simulink model "v5_2025_11_26_D2_rate_adaptive_revised"  (R2025a)
settings: Solver=FixedStepAuto  StartTime=0.0  StopTime=inf  FixedStep=1e-3  RelTol=1e-3  EnableMultiTasking=on
undefined symbols (not defined in the file): A0, A1, D0, D1, D10, D11, D12, D13, D2, D3, D4, D5, D6, D7, D8, D9, PTA0, PTA1, PTA2, PTB2, PTB23, PTB3, PTB9, PTC16, PTC17, PTC2, PTC3, PTC4, PTD0, PTD1, PTD2, PTD3
libraries: frdmk64flib x18, etargetslib x2, dspstat3 x1
settings Model: ExtModeTrigDuration=5  Creator=School Account  LastModifiedBy=zhang
settings SolverCC: AlgebraicLoopSolver=TrustRegion
settings OptimizationCC: DefaultParameterBehavior=Inlined  EnhancedBackFolding=on  PassReuseOutputArgsAs=Individual arguments  ZeroExternalMemoryAtStartup=off  ZeroInternalMemoryAtStartup=off  MaxStackSize=64  OptimizeBlockOrder=speed  DifferentSizesBufferReuse=on  OptimizationCustomize=off  EfficientTunableParamExpr=on
settings DebuggingCC: ParameterTunabilityLossMsg=error
settings HardwareCC: ProdBitPerPointer=32.0  ProdBitPerSizeT=32.0  ProdBitPerPtrDiffT=32.0  ProdLargestAtomicInteger=Long  ProdLargestAtomicFloat=Double  ProdWordSize=32.0  ProdHWDeviceType=ARM Compatible->ARM Cortex
settings SFSimCC: MATLABDynamicMemAlloc=off
settings RTWCC: SystemTargetFile=ert.tlc  HardwareBoard=NXP FRDM-K64F  TLCOptions="-aInlineSetEventsForThisBaseRateFcn=TLC_FALSE -aSuppressMultiTaskScheduler=TLC_FALSE  -aRateBasedStepFcn=0"  TemplateMakefile=ert_default_tmf  Toolchain=GNU Tools for ARM Embedded Processors  GPUComputeCapability=3.5  Description=Embedded Coder
settings CodeAppCC: ForceParamTrailComments=on  IgnoreCustomStorageClasses=off  OperatorAnnotations=on  SimulinkDataObjDesc=on  SFDataObjDesc=on  InsertBlockDesc=on
settings ERTTargetCC: ExtModeTransport=4.0  ExtModeStaticAlloc=off  ExtModeMexFile=sendToCommService  ExtModeIntrfLevel=Level1  DynamicArrayContainerType=coder::array

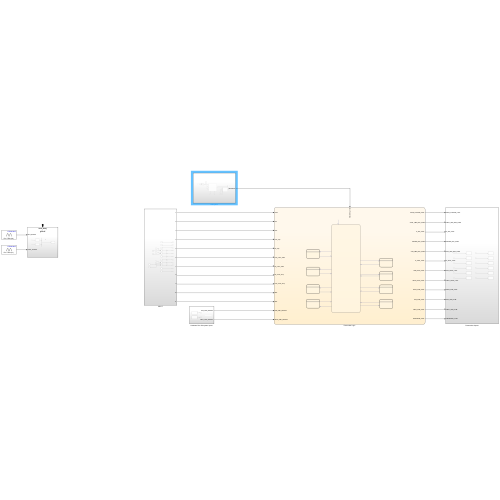
[thumbnail: Simulink's stored preview of the top-level diagram]
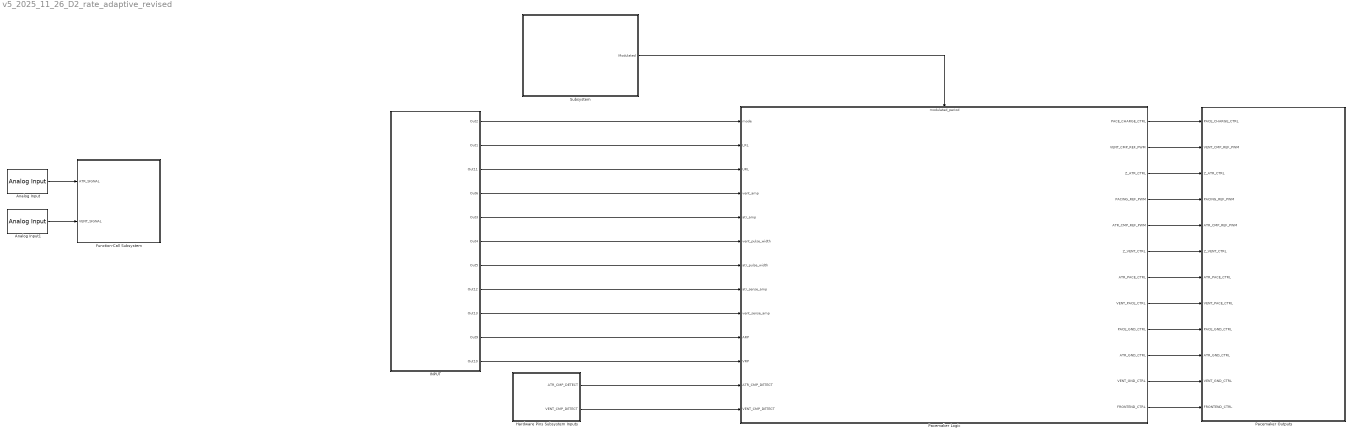
== system v5_2025_11_26_D2_rate_adaptive_revised ==
  Analog Input : frdmk64flib/Analog Input  Whichpin=PTB2 (A0)  SampleTime=-1
  Analog Input1 : frdmk64flib/Analog Input  Whichpin=PTB3 (A1)  SampleTime=-1
  Function-Call Subsystem : Subsystem  TreatAsAtomicUnit=on
  Hardware Pins Subsystem Inputs : Subsystem
  "INPUT " : Subsystem
  Pacemaker Logic : Stateflow chart  TreatAsAtomicUnit=on
      settings: PortSchema="{\"entries\":[{\"content\":{\"sides\":[{\"content\":{\"connectorIds\":[\"In1\",\"In4\",\"In13\",\"In5\",\"In2\",\"In6\",\"In3\",\"In7\",\"In10\",\"In8\",\"In11\",\"In9\",\"In12\"]},\"type\":\"ConnectorPlacement.EquallySpacedRectSide\",\"uuid\":\"2821f65a-9b3e-4ca7-babd-b0602bfdca31\"},{\"content\":{\"connectorIds\":[\"Out1\",\"Out2\",\"Out3\",\"Out4\",\"Out5\",\"Out6\",\"Out7\",\"Out8\",\"Out9\",\"Out10\",\"Out11\",\"Out12\"],\"side\":\"RIGHT\"},\"type\":\"ConnectorPlacement.EquallySpacedRectSide\",\"uuid\":\"3302ad84-7e85-4bae-9388-240b69681e7f\"},{\"content\":{\"connectorIds\":[\"In14\"],\"side\":\"TOP\"},\"type\":\"ConnectorPlacement.EquallySpacedRectSide\",\"uuid\":\"cc666da6-1c79-42dc-9f95-9791247ae8bf\"},{\"content\":{\"side\":\"BOTTOM\"},\"type\":\"ConnectorPlacement.EquallySpacedRectSide\",\"uuid\":\"6c7eefe5-bab4-42c2-8766-4f3cee9532f0\"}]},\"type\":\"ConnectorPlacement.EquallySpacedConnector\",\"uuid\":\"e2a43bfa-d126-4f35-adbf-2cf33da0501f\"}],\"packageUris\":[\"http://schema.mathworks.com/mf0/Connector/R2020b\"],\"version\":\"1.0\"}"
  Pacemaker Outputs : Subsystem
  Subsystem : Subsystem
  wires:
  Pacemaker Logic/1(PACE_CHARGE_CTRL) -> Pacemaker Outputs/1(PACE_CHARGE_CTRL)
  Pacemaker Logic/3(Z_ATR_CTRL) -> Pacemaker Outputs/3(Z_ATR_CTRL)
  Pacemaker Logic/4(PACING_REF_PWM) -> Pacemaker Outputs/4(PACING_REF_PWM)
  Pacemaker Logic/7(ATR_PACE_CTRL) -> Pacemaker Outputs/7(ATR_PACE_CTRL)
  Pacemaker Logic/9(PACE_GND_CTRL) -> Pacemaker Outputs/9(PACE_GND_CTRL)
  Pacemaker Logic/10(ATR_GND_CTRL) -> Pacemaker Outputs/10(ATR_GND_CTRL)
  Pacemaker Logic/11(VENT_GND_CTRL) -> Pacemaker Outputs/11(VENT_GND_CTRL)
  Pacemaker Logic/8(VENT_PACE_CTRL) -> Pacemaker Outputs/8(VENT_PACE_CTRL)
  Pacemaker Logic/6(Z_VENT_CTRL) -> Pacemaker Outputs/6(Z_VENT_CTRL)
  Pacemaker Logic/12(FRONTEND_CTRL) -> Pacemaker Outputs/12(FRONTEND_CTRL)
  Pacemaker Logic/5(ATR_CMP_REF_PWM) -> Pacemaker Outputs/5(ATR_CMP_REF_PWM)
  Pacemaker Logic/2(VENT_CMP_REF_PWM) -> Pacemaker Outputs/2(VENT_CMP_REF_PWM)
  Hardware Pins Subsystem Inputs/2(VENT_CMP_DETECT) -> Pacemaker Logic/12(VENT_CMP_DETECT)
  Hardware Pins Subsystem Inputs/1(ATR_CMP_DETECT) -> Pacemaker Logic/9(ATR_CMP_DETECT)
  "INPUT "/10(Out9) -> Pacemaker Logic/8(ARP)
  "INPUT "/11(Out10) -> Pacemaker Logic/11(VRP)
  "INPUT "/9(Out13) -> Pacemaker Logic/10(vent_sense_amp)
  "INPUT "/8(Out12) -> Pacemaker Logic/7(atr_sense_amp)
  "INPUT "/7(Out5) -> Pacemaker Logic/3(atr_pulse_width)
  "INPUT "/6(Out4) -> Pacemaker Logic/6(vent_pulse_width)
  "INPUT "/5(Out3) -> Pacemaker Logic/2(atr_amp)
  "INPUT "/4(Out6) -> Pacemaker Logic/5(vent_amp)
  "INPUT "/1(Out2) -> Pacemaker Logic/1(mode)
  "INPUT "/2(Out1) -> Pacemaker Logic/4(LRL)
  "INPUT "/3(Out11) -> Pacemaker Logic/13(URL)
  Analog Input/1 -> Function-Call Subsystem/1(ATR_SIGNAL)
  Analog Input1/1 -> Function-Call Subsystem/2(VENT_SIGNAL)
  Subsystem/1(Modulated) -> Pacemaker Logic/14(modulated_period)

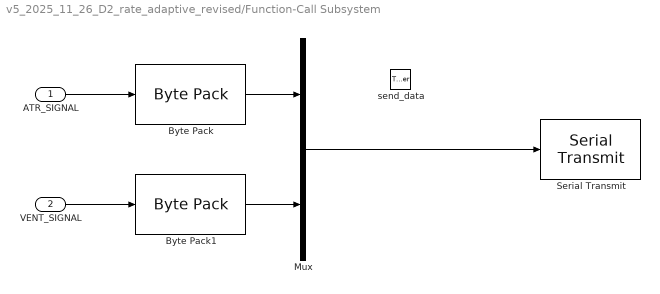
== system v5_2025_11_26_D2_rate_adaptive_revised/Function-Call Subsystem ==
  ATR_SIGNAL : Inport
  VENT_SIGNAL : Inport  Port=2
  send_data : TriggerPort  TriggerType=function-call  IsSimulinkFunction=on  FunctionName=send_data  VariantControl=(inherit)
  Byte Pack : etargetslib/Byte Pack  datatypes={'double'}  byteAlign=1
  Byte Pack1 : etargetslib/Byte Pack  datatypes={'double'}  byteAlign=1
  Mux : Mux  Inputs=2
  Serial Transmit : frdmk64flib/Serial Transmit  SCIModule=0  Baudrate=uint32(9600)  Parity=None  StopBits=1  HardwareFlowControl=None  ByteOrder=LittleEndian  BlockingMode=on  OutputStatus=off
  wires:
  ATR_SIGNAL/1 -> Byte Pack/1
  VENT_SIGNAL/1 -> Byte Pack1/1
  Byte Pack/1 -> Mux/1
  Mux/1 -> Serial Transmit/1
  Byte Pack1/1 -> Mux/2

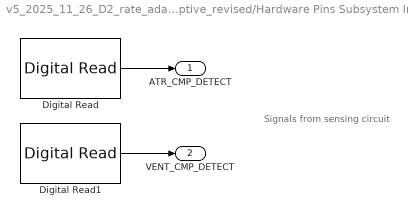
== system v5_2025_11_26_D2_rate_adaptive_revised/Hardware Pins Subsystem Inputs ==
  note: Signals from sensing circuit
  Digital Read : frdmk64flib/Digital Read  Whichpin=PTC16 (D0)  SampleTime=-1
  Digital Read1 : frdmk64flib/Digital Read  Whichpin=PTC17 (D1)  SampleTime=-1
  ATR_CMP_DETECT : Outport
  VENT_CMP_DETECT : Outport  Port=2
  wires:
  Digital Read1/1 -> VENT_CMP_DETECT/1
  Digital Read/1 -> ATR_CMP_DETECT/1

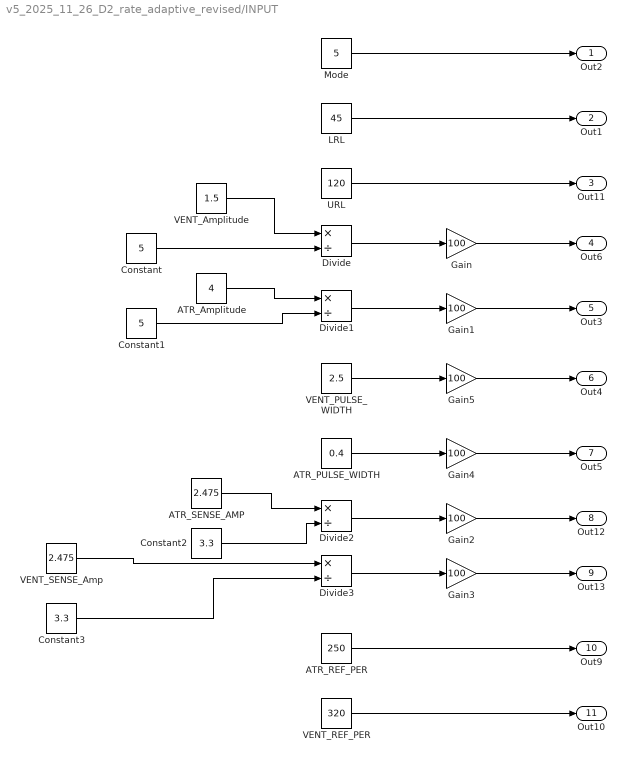
== system v5_2025_11_26_D2_rate_adaptive_revised/INPUT  ==
  ATR_Amplitude : Constant  Value=4
  ATR_PULSE_WIDTH : Constant  Value=0.4
  ATR_REF_PER : Constant  Value=250
  ATR_SENSE_AMP : Constant  Value=2.475
  Constant : Constant  Value=5
  Constant1 : Constant  Value=5
  Constant2 : Constant  Value=3.3
  Constant3 : Constant  Value=3.3
  Divide{,1..3} (4 alike) : Product  Inputs=*/
  Gain{,1..5} (6 alike) : Gain  Gain=100
  LRL : Constant  Value=45
  Mode : Constant  Value=5
  URL : Constant  Value=120
  VENT_Amplitude : Constant  Value=1.5
  VENT_PULSE_WIDTH : Constant  Value=2.5
  VENT_REF_PER : Constant  Value=320
  VENT_SENSE_Amp : Constant  Value=2.475
  Out2 : Outport
  Out1 : Outport  Port=2
  Out11 : Outport  Port=3
  Out6 : Outport  Port=4
  Out3 : Outport  Port=5
  Out4 : Outport  Port=6
  Out5 : Outport  Port=7
  Out12 : Outport  Port=8
  Out13 : Outport  Port=9
  Out9 : Outport  Port=10
  Out10 : Outport  Port=11
  wires:
  LRL/1 -> Out1/1
  URL/1 -> Out11/1
  Mode/1 -> Out2/1
  ATR_REF_PER/1 -> Out9/1
  VENT_REF_PER/1 -> Out10/1
  VENT_Amplitude/1 -> Divide/1
  Gain/1 -> Out6/1
  ATR_Amplitude/1 -> Divide1/1
  Gain1/1 -> Out3/1
  ATR_SENSE_AMP/1 -> Divide2/1
  Gain2/1 -> Out12/1
  VENT_SENSE_Amp/1 -> Divide3/1
  Gain3/1 -> Out13/1
  VENT_PULSE_WIDTH/1 -> Gain5/1
  Gain5/1 -> Out4/1
  ATR_PULSE_WIDTH/1 -> Gain4/1
  Gain4/1 -> Out5/1
  Divide/1 -> Gain/1
  Constant/1 -> Divide/2
  Divide1/1 -> Gain1/1
  Constant1/1 -> Divide1/2
  Divide2/1 -> Gain2/1
  Constant2/1 -> Divide2/2
  Divide3/1 -> Gain3/1
  Constant3/1 -> Divide3/2

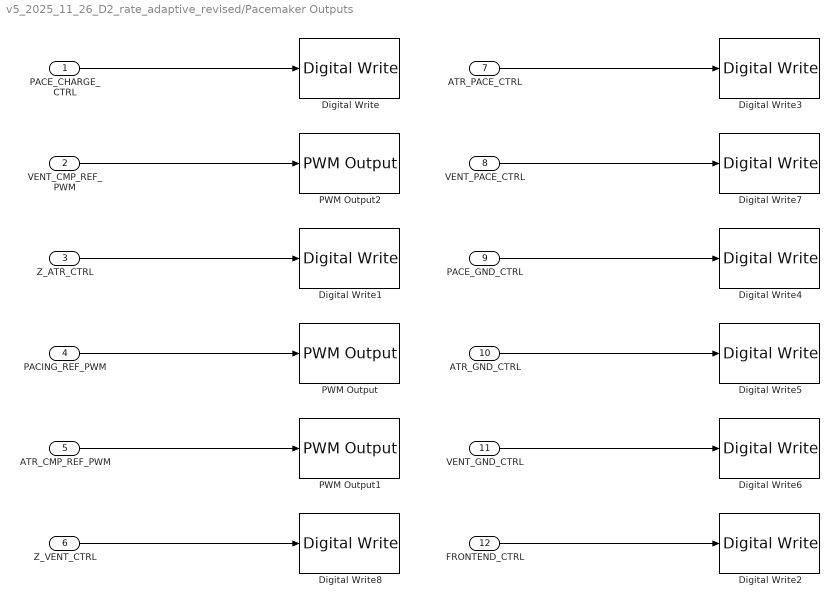
== system v5_2025_11_26_D2_rate_adaptive_revised/Pacemaker Outputs ==
  PACE_CHARGE_CTRL : Inport
  VENT_CMP_REF_PWM : Inport  Port=2
  Z_ATR_CTRL : Inport  Port=3
  PACING_REF_PWM : Inport  Port=4
  ATR_CMP_REF_PWM : Inport  Port=5
  Z_VENT_CTRL : Inport  Port=6
  ATR_PACE_CTRL : Inport  Port=7
  VENT_PACE_CTRL : Inport  Port=8
  PACE_GND_CTRL : Inport  Port=9
  ATR_GND_CTRL : Inport  Port=10
  VENT_GND_CTRL : Inport  Port=11
  FRONTEND_CTRL : Inport  Port=12
  Digital Write : frdmk64flib/Digital Write  Whichpin=PTB9 (D2)
  Digital Write1 : frdmk64flib/Digital Write  Whichpin=PTB23 (D4)
  Digital Write2 : frdmk64flib/Digital Write  Whichpin=PTD1 (D13)
  Digital Write3 : frdmk64flib/Digital Write  Whichpin=PTA0 (D8)
  Digital Write4 : frdmk64flib/Digital Write  Whichpin=PTD0 (D10)
  Digital Write5 : frdmk64flib/Digital Write  Whichpin=PTD2 (D11)
  Digital Write6 : frdmk64flib/Digital Write  Whichpin=PTD3 (D12)
  Digital Write7 : frdmk64flib/Digital Write  Whichpin=PTC4 (D9)
  Digital Write8 : frdmk64flib/Digital Write  Whichpin=PTC3 (D7)
  PWM Output : frdmk64flib/PWM Output  Whichpin=PTA2 (D5)  InitialFrequency=2000  InitialDutyCycle=0
  PWM Output1 : frdmk64flib/PWM Output  Whichpin=PTC2 (D6)  InitialFrequency=2000  InitialDutyCycle=0
  PWM Output2 : frdmk64flib/PWM Output  Whichpin=PTA1 (D3)  InitialFrequency=2000  InitialDutyCycle=0
  wires:
  PACE_CHARGE_CTRL/1 -> Digital Write/1
  Z_ATR_CTRL/1 -> Digital Write1/1
  PACING_REF_PWM/1 -> PWM Output/1
  ATR_PACE_CTRL/1 -> Digital Write3/1
  PACE_GND_CTRL/1 -> Digital Write4/1
  ATR_GND_CTRL/1 -> Digital Write5/1
  VENT_GND_CTRL/1 -> Digital Write6/1
  VENT_PACE_CTRL/1 -> Digital Write7/1
  Z_VENT_CTRL/1 -> Digital Write8/1
  FRONTEND_CTRL/1 -> Digital Write2/1
  ATR_CMP_REF_PWM/1 -> PWM Output1/1
  VENT_CMP_REF_PWM/1 -> PWM Output2/1

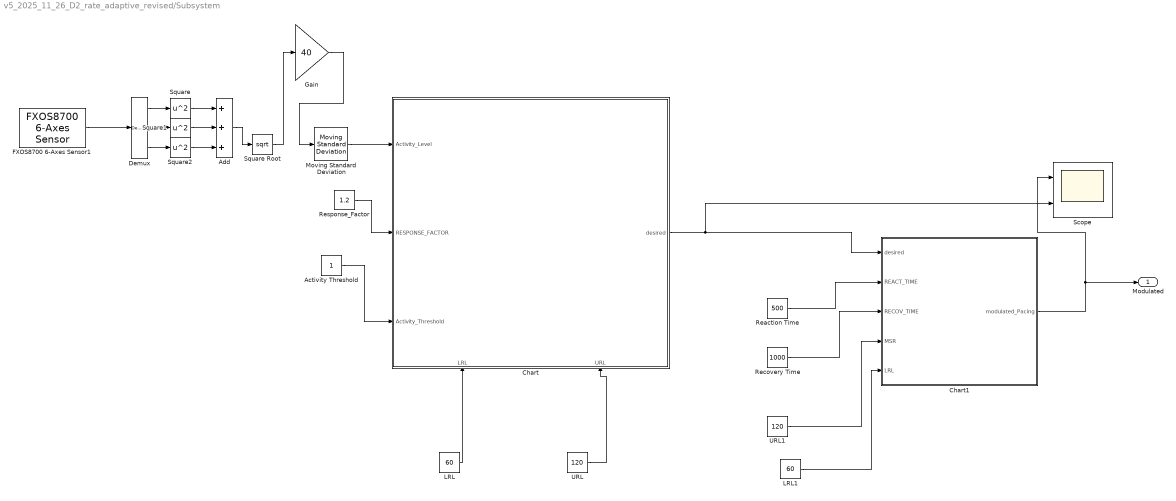
== system v5_2025_11_26_D2_rate_adaptive_revised/Subsystem ==
  Activity Threshold : Constant
  Add : Sum  Inputs=+++
  Chart : Stateflow chart  TreatAsAtomicUnit=on
      settings: PortSchema="{\"entries\":[{\"content\":{\"sides\":[{\"content\":{\"connectorIds\":[\"In3\",\"In4\",\"In5\"]},\"type\":\"ConnectorPlacement.EquallySpacedRectSide\",\"uuid\":\"74c786d3-d2a6-437e-8bb7-c9d9b4a74617\"},{\"content\":{\"connectorIds\":[\"Out1\"],\"side\":\"RIGHT\"},\"type\":\"ConnectorPlacement.EquallySpacedRectSide\",\"uuid\":\"2c46704d-1ce5-4a26-9635-57e0f6503ead\"},{\"content\":{\"side\":\"TOP\"},\"type\":\"ConnectorPlacement.EquallySpacedRectSide\",\"uuid\":\"1e7c0bb1-a8b6-49e0-9e63-e8e48adc5546\"},{\"content\":{\"connectorIds\":[\"In1\",\"In2\"],\"side\":\"BOTTOM\"},\"type\":\"ConnectorPlacement.EquallySpacedRectSide\",\"uuid\":\"98fe2a4d-8dd5-42bc-97d4-b5234350e537\"}]},\"type\":\"ConnectorPlacement.EquallySpacedConnector\",\"uuid\":\"114a6ead-843c-4291-bcbc-4dc58f15d580\"}],\"packageUris\":[\"http://schema.mathworks.com/mf0/Connector/R2020b\"],\"version\":\"1.0\"}"
  Chart1 : Stateflow chart  TreatAsAtomicUnit=on
  Demux : Demux  Outputs=3
  FXOS8700 6-Axes Sensor1 : frdmk64flib/FXOS8700 6-Axes Sensor  Activesensor=Accelerometer only  ODR=800Hz  HybridODR=400Hz  Accelfullrange=-4g to +4g  SampleTime=0.01
  Gain : Gain  Gain=40
  LRL : Constant  Value=60
  LRL1 : Constant  Value=60
  Moving Standard Deviation : dspstat3/Moving Standard Deviation  Method=Sliding window  ForgettingFactorPort=off  SpecifyWindowLength=on  WindowLength=128  OverlapLength=127  AllowArbitraryInputLength=off  ForgettingFactor=0.9  SimulateUsing=Interpreted execution
  Reaction Time : Constant  Value=500
  Recovery Time : Constant  Value=1000
  Response_Factor : Constant  Value=1.2
  Scope : Scope  NumInputPorts=2
      settings: ActiveDisplayYMinimum=-63.251795567262889  ActiveDisplayYMaximum=284.31092337041139
  Square : Math  Operator=square
  Square Root : Sqrt
  Square1 : Math  Operator=square
  Square2 : Math  Operator=square
  URL : Constant  Value=120
  URL1 : Constant  Value=120
  Modulated : Outport
  wires:
  Square1/1 -> Add/2
  Demux/1 -> Square/1
  Square2/1 -> Add/3
  Square/1 -> Add/1
  Demux/2 -> Square1/1
  Demux/3 -> Square2/1
  Add/1 -> Square Root/1
  FXOS8700 6-Axes Sensor1/1 -> Demux/1
  Activity Threshold/1 -> Chart/5(Activity_Threshold)
  Response_Factor/1 -> Chart/4(RESPONSE_FACTOR)
  Reaction Time/1 -> Chart1/2(REACT_TIME)
  Recovery Time/1 -> Chart1/3(RECOV_TIME)
  Chart1/1(modulated_Pacing) -> Modulated/1, Scope/1
  LRL/1 -> Chart/1(LRL)
  URL/1 -> Chart/2(URL)
  URL1/1 -> Chart1/4(MSR)
  LRL1/1 -> Chart1/5(LRL)
  Chart/1(desired) -> Chart1/1(desired), Scope/2
  Moving Standard Deviation/1 -> Chart/3(Activity_Level)
  Square Root/1 -> Gain/1
  Gain/1 -> Moving Standard Deviation/1

== stateflow chart v5_2025_11_26_D2_rate_adaptive_revised/Subsystem/Chart ==
  state UpperLimiter [commented out]
    entry:
    desired = URL
  state LinearFunction
    during:
    desired = RESPONSE_FACTOR * (Activity_Level  -  Activity_Threshold) + LRL
    % 2. Apply Upper Limit (Clamp to URL)
    if desired > URL
    desired = URL;
    % 3. Apply Lower Limit (Clamp to LRL)
    elseif desired < LRL
    desired = LRL;
    end
  state Init
    entry:
    desired = LRL
  state Start
  state LowerLimiter [commented out]
    entry:
    desired = LRL
  LinearFunction -> UpperLimiter [commented out] : [desired > URL]
  UpperLimiter -> LinearFunction [commented out] : [desired <= URL]
  (default) -> Init
  Init -> Start
  Start -> LinearFunction : [Activity_Level >= Activity_Threshold]
  LinearFunction -> Start : [Activity_Level < Activity_Threshold]
  LowerLimiter -> LinearFunction [commented out] : [desired >= LRL]
  LinearFunction -> LowerLimiter [commented out] : [desired < LRL]
  data: LRL input; URL input; Activity_Level input; RESPONSE_FACTOR input; Activity_Threshold input; desired output

== stateflow chart v5_2025_11_26_D2_rate_adaptive_revised/Subsystem/Chart1 ==
  state Pacing_Up
    during:
    % Calculate the step size needed to close the gap based on REACT_TIME
    % Doing this every step creates a smooth approach
    increment = (desired - modulated_Pacing) / REACT_TIME;
    % Apply the increment (assuming 1ms step)
    modulated_Pacing = modulated_Pacing + increment;
    % Safety Clamp: Don't go over MSR
    if modulated_Pacing > MSR
    modulated_Pacing = MSR;
    end
  state Steady_State
    during:
    difference=desired - modulated_Pacing
  state Init1
    entry:
    modulated_Pacing=LRL
  state Pacing_Down
    during:
    % Calculate the decrement based on RECOV_TIME
    decrement = (desired - modulated_Pacing) / RECOV_TIME;
    % Note: decrement will be negative because (desired - modulated) is negative
    % Apply the decrement
    modulated_Pacing = modulated_Pacing + decrement;
    % Safety Clamp: Don't go under LRL
    if modulated_Pacing < LRL
    modulated_Pacing = LRL;
    end
  Steady_State -> Pacing_Up [order 1] : [desired > modulated_Pacing]
  Pacing_Up -> Steady_State : [modulated_Pacing >= desired]
  Init1 -> Steady_State
  Steady_State -> Pacing_Down [order 2] : [desired < modulated_Pacing]
  Pacing_Down -> Steady_State : [modulated_Pacing <= desired]
  (default) -> Init1
  data: desired input; REACT_TIME input; RECOV_TIME input; modulated_Pacing output =60; difference local; increment local; decrement local; MSR input; LRL input

== stateflow chart v5_2025_11_26_D2_rate_adaptive_revised/Pacemaker Logic ==
  state Start
  state VVIR
    state VVI_Charge
      entry:
      FRONTEND_CTRL = 1;
      %Charging C22
      VENT_PACE_CTRL = 0;
      ATR_PACE_CTRL = 0;
      PACING_REF_PWM = vent_amp;
      PACE_CHARGE_CTRL = 1;
      %Discharging C21
      PACE_GND_CTRL = 1;
      VENT_PACE_CTRL = 0;
      Z_ATR_CTRL = 0;
      Z_VENT_CTRL = 0;
      ATR_PACE_CTRL = 0;
      ATR_GND_CTRL = 0;
      VENT_GND_CTRL = 1;
      VENT_CMP_REF_PWM = vent_sense_amp;
    state VVI_Pace
      entry:
      %Pacing
      PACE_CHARGE_CTRL = 0;
      PACE_GND_CTRL= 1;
      ATR_PACE_CTRL = 0;
      ATR_GND_CTRL= 0;
      Z_ATR_CTRL = 0;
      Z_VENT_CTRL = 0;
      VENT_GND_CTRL = 0;
      VENT_PACE_CTRL = 1;
    state VVI_Inhibit
      entry:
      FRONTEND_CTRL = 0;
      %Charging C22
      VENT_PACE_CTRL = 0;
      ATR_PACE_CTRL = 0;
      PACING_REF_PWM = vent_amp;
      PACE_CHARGE_CTRL = 1;
      %Discharging C21
      PACE_GND_CTRL = 1;
      VENT_PACE_CTRL = 0;
      Z_VENT_CTRL = 0;
      Z_ATR_CTRL = 0;
      ATR_PACE_CTRL = 0;
      ATR_GND_CTRL = 0;
      VENT_GND_CTRL = 1;
      VENT_CMP_REF_PWM = vent_sense_amp;
    (default) -> VVIR.VVI_Charge
    VVIR.VVI_Charge -> VVIR.VVI_Pace [order 1] : [after(60000/modulated_period - vent_pulse_width - VRP,msec)]
    VVIR.VVI_Charge -> (junction 112) [order 2] : [VENT_CMP_DETECT == 1]
    (junction 112) -> VVIR.VVI_Inhibit : [after(60000/modulated_period - VRP,msec)]
    VVIR.VVI_Pace -> VVIR.VVI_Inhibit : [after(vent_pulse_width,msec)]
    VVIR.VVI_Inhibit -> VVIR.VVI_Charge : [after(VRP, msec)]
  state VVI
    state VVI_Charge
      entry:
      FRONTEND_CTRL = 1;
      %Charging C22
      VENT_PACE_CTRL = 0;
      ATR_PACE_CTRL = 0;
      PACING_REF_PWM = vent_amp;
      PACE_CHARGE_CTRL = 1;
      %Discharging C21
      PACE_GND_CTRL = 1;
      VENT_PACE_CTRL = 0;
      Z_ATR_CTRL = 0;
      Z_VENT_CTRL = 0;
      ATR_PACE_CTRL = 0;
      ATR_GND_CTRL = 0;
      VENT_GND_CTRL = 1;
      VENT_CMP_REF_PWM = vent_sense_amp;
    state VVI_Pace
      entry:
      %Pacing
      PACE_CHARGE_CTRL = 0;
      PACE_GND_CTRL= 1;
      ATR_PACE_CTRL = 0;
      ATR_GND_CTRL= 0;
      Z_ATR_CTRL = 0;
      Z_VENT_CTRL = 0;
      VENT_GND_CTRL = 0;
      VENT_PACE_CTRL = 1;
    state VVI_Inhibit
      entry:
      FRONTEND_CTRL = 0;
      %Charging C22
      VENT_PACE_CTRL = 0;
      ATR_PACE_CTRL = 0;
      PACING_REF_PWM = vent_amp;
      PACE_CHARGE_CTRL = 1;
      %Discharging C21
      PACE_GND_CTRL = 1;
      VENT_PACE_CTRL = 0;
      Z_VENT_CTRL = 0;
      Z_ATR_CTRL = 0;
      ATR_PACE_CTRL = 0;
      ATR_GND_CTRL = 0;
      VENT_GND_CTRL = 1;
      VENT_CMP_REF_PWM = vent_sense_amp;
    (default) -> VVI.VVI_Charge
    VVI.VVI_Charge -> VVI.VVI_Pace [order 1] : [after(60000/LRL - vent_pulse_width - VRP,msec)]
    VVI.VVI_Charge -> (junction 65) [order 2] : [VENT_CMP_DETECT == 1]
    (junction 65) -> VVI.VVI_Inhibit : [after(60000/LRL - VRP,msec)]
    VVI.VVI_Pace -> VVI.VVI_Inhibit : [after(vent_pulse_width,msec)]
    VVI.VVI_Inhibit -> VVI.VVI_Charge : [after(VRP, msec)]
  state AAIR
    state AAI_Charge
      entry:
      FRONTEND_CTRL = 1;
      %Charging C22
      ATR_PACE_CTRL = 0;
      VENT_PACE_CTRL = 0;
      PACING_REF_PWM = atr_amp;
      PACE_CHARGE_CTRL = 1;
      %Discharging C21
      PACE_GND_CTRL = 1;
      ATR_PACE_CTRL = 0;
      Z_VENT_CTRL = 0;
      Z_ATR_CTRL = 0;
      VENT_PACE_CTRL = 0;
      VENT_GND_CTRL = 0;
      ATR_GND_CTRL = 1;
      ATR_CMP_REF_PWM = atr_sense_amp;
    state AAI_Pace
      entry:
      %Pacing
      PACE_CHARGE_CTRL = 0;
      PACE_GND_CTRL= 1;
      VENT_PACE_CTRL = 0;
      VENT_GND_CTRL= 0;
      Z_VENT_CTRL = 0;
      Z_ATR_CTRL = 0;
      ATR_GND_CTRL = 0;
      ATR_PACE_CTRL = 1;
    state AAI_Inhibit
      entry:
      FRONTEND_CTRL = 0;
      %Charging C22
      ATR_PACE_CTRL = 0;
      VENT_PACE_CTRL = 0;
      PACING_REF_PWM = atr_amp;
      PACE_CHARGE_CTRL = 1;
      %Discharging C21
      PACE_GND_CTRL = 1;
      ATR_PACE_CTRL = 0;
      Z_VENT_CTRL = 0;
      Z_ATR_CTRL = 0;
      VENT_PACE_CTRL = 0;
      VENT_GND_CTRL = 0;
      ATR_GND_CTRL = 1;
      ATR_CMP_REF_PWM = atr_sense_amp;
    (default) -> AAIR.AAI_Charge
    AAIR.AAI_Charge -> AAIR.AAI_Pace [order 1] : [after(60000/modulated_period - atr_pulse_width - ARP,msec)]
    AAIR.AAI_Charge -> (junction 101) [order 2] : [ATR_CMP_DETECT == 1]
    (junction 101) -> AAIR.AAI_Inhibit : [after(60000/modulated_period - ARP,msec)]
    AAIR.AAI_Pace -> AAIR.AAI_Inhibit : [after(atr_pulse_width,msec)]
    AAIR.AAI_Inhibit -> AAIR.AAI_Charge : [after(ARP, msec)]
  state AAI
    state AAI_Charge
      entry:
      FRONTEND_CTRL = 1;
      %Charging C22
      ATR_PACE_CTRL = 0;
      VENT_PACE_CTRL = 0;
      PACING_REF_PWM = atr_amp;
      PACE_CHARGE_CTRL = 1;
      %Discharging C21
      PACE_GND_CTRL = 1;
      ATR_PACE_CTRL = 0;
      Z_VENT_CTRL = 0;
      Z_ATR_CTRL = 0;
      VENT_PACE_CTRL = 0;
      VENT_GND_CTRL = 0;
      ATR_GND_CTRL = 1;
      ATR_CMP_REF_PWM = atr_sense_amp;
    state AAI_Pace
      entry:
      %Pacing
      PACE_CHARGE_CTRL = 0;
      PACE_GND_CTRL= 1;
      VENT_PACE_CTRL = 0;
      VENT_GND_CTRL= 0;
      Z_VENT_CTRL = 0;
      Z_ATR_CTRL = 0;
      ATR_GND_CTRL = 0;
      ATR_PACE_CTRL = 1;
    state AAI_Inhibit
      entry:
      FRONTEND_CTRL = 0;
      %Charging C22
      ATR_PACE_CTRL = 0;
      VENT_PACE_CTRL = 0;
      PACING_REF_PWM = atr_amp;
      PACE_CHARGE_CTRL = 1;
      %Discharging C21
      PACE_GND_CTRL = 1;
      ATR_PACE_CTRL = 0;
      Z_VENT_CTRL = 0;
      Z_ATR_CTRL = 0;
      VENT_PACE_CTRL = 0;
      VENT_GND_CTRL = 0;
      ATR_GND_CTRL = 1;
      ATR_CMP_REF_PWM = atr_sense_amp;
    (default) -> AAI.AAI_Charge
    AAI.AAI_Charge -> AAI.AAI_Pace [order 1] : [after(60000/LRL - atr_pulse_width - ARP,msec)]
    AAI.AAI_Charge -> (junction 58) [order 2] : [ATR_CMP_DETECT == 1]
    (junction 58) -> AAI.AAI_Inhibit : [after(60000/LRL - ARP,msec)]
    AAI.AAI_Pace -> AAI.AAI_Inhibit : [after(atr_pulse_width,msec)]
    AAI.AAI_Inhibit -> AAI.AAI_Charge : [after(ARP, msec)]
  state VOOR
    state VOO_Charge
      entry:
      %Charging C22
      VENT_PACE_CTRL = 0;
      ATR_PACE_CTRL = 0;
      PACING_REF_PWM = vent_amp;
      PACE_CHARGE_CTRL = 1;
      %Discharging C21
      PACE_GND_CTRL = 1;
      VENT_PACE_CTRL = 0;
      Z_ATR_CTRL = 0;
      Z_VENT_CTRL = 0;
      ATR_PACE_CTRL = 0;
      ATR_GND_CTRL = 0;
      VENT_GND_CTRL = 1;
    state AOO_Pace
      entry:
      %Pacing
      PACE_CHARGE_CTRL = 0;
      PACE_GND_CTRL= 1;
      ATR_PACE_CTRL = 0;
      ATR_GND_CTRL= 0;
      Z_ATR_CTRL = 0;
      Z_VENT_CTRL = 0;
      VENT_GND_CTRL = 0;
      VENT_PACE_CTRL = 1;
    (default) -> VOOR.VOO_Charge
    VOOR.VOO_Charge -> VOOR.AOO_Pace : [after(60000/modulated_period - vent_pulse_width,msec)]
    VOOR.AOO_Pace -> VOOR.VOO_Charge : [after(vent_pulse_width,msec)]
  state VOO
    state VOO_Charge
      entry:
      %Charging C22
      VENT_PACE_CTRL = 0;
      ATR_PACE_CTRL = 0;
      PACING_REF_PWM = vent_amp;
      PACE_CHARGE_CTRL = 1;
      %Discharging C21
      PACE_GND_CTRL = 1;
      VENT_PACE_CTRL = 0;
      Z_ATR_CTRL = 0;
      Z_VENT_CTRL = 0;
      ATR_PACE_CTRL = 0;
      ATR_GND_CTRL = 0;
      VENT_GND_CTRL = 1;
    state AOO_Pace
      entry:
      %Pacing
      PACE_CHARGE_CTRL = 0;
      PACE_GND_CTRL= 1;
      ATR_PACE_CTRL = 0;
      ATR_GND_CTRL= 0;
      Z_ATR_CTRL = 0;
      Z_VENT_CTRL = 0;
      VENT_GND_CTRL = 0;
      VENT_PACE_CTRL = 1;
    (default) -> VOO.VOO_Charge
    VOO.VOO_Charge -> VOO.AOO_Pace : [after(60000/LRL - vent_pulse_width,msec)]
    VOO.AOO_Pace -> VOO.VOO_Charge : [after(vent_pulse_width,msec)]
  state AOOR
    state AOO_Charge
      entry:
      %Charging C22
      ATR_PACE_CTRL = 0;
      VENT_PACE_CTRL = 0;
      PACING_REF_PWM = atr_amp;
      PACE_CHARGE_CTRL = 1;
      %Discharging C21
      PACE_GND_CTRL = 1;
      ATR_PACE_CTRL = 0;
      Z_VENT_CTRL = 0;
      Z_ATR_CTRL = 0;
      VENT_PACE_CTRL = 0;
      VENT_GND_CTRL = 0;
      ATR_GND_CTRL = 1;
    state AOO_Pace
      entry:
      %Pacing
      PACE_CHARGE_CTRL = 0;
      PACE_GND_CTRL= 1;
      VENT_PACE_CTRL = 0;
      VENT_GND_CTRL= 0;
      Z_VENT_CTRL = 0;
      Z_ATR_CTRL = 0;
      ATR_GND_CTRL = 0;
      ATR_PACE_CTRL = 1;
    (default) -> AOOR.AOO_Charge
    AOOR.AOO_Charge -> AOOR.AOO_Pace : [after(60000/modulated_period - atr_pulse_width,msec)]
    AOOR.AOO_Pace -> AOOR.AOO_Charge : [after(atr_pulse_width,msec)]
  state AOO
    state AOO_Charge
      entry:
      %Charging C22
      ATR_PACE_CTRL = 0;
      VENT_PACE_CTRL = 0;
      PACING_REF_PWM = atr_amp;
      PACE_CHARGE_CTRL = 1;
      %Discharging C21
      PACE_GND_CTRL = 1;
      ATR_PACE_CTRL = 0;
      Z_VENT_CTRL = 0;
      Z_ATR_CTRL = 0;
      VENT_PACE_CTRL = 0;
      VENT_GND_CTRL = 0;
      ATR_GND_CTRL = 1;
    state AOO_Pace
      entry:
      %Pacing
      PACE_CHARGE_CTRL = 0;
      PACE_GND_CTRL= 1;
      VENT_PACE_CTRL = 0;
      VENT_GND_CTRL= 0;
      Z_VENT_CTRL = 0;
      Z_ATR_CTRL = 0;
      ATR_GND_CTRL = 0;
      ATR_PACE_CTRL = 1;
    (default) -> AOO.AOO_Charge
    AOO.AOO_Charge -> AOO.AOO_Pace : [after(60000/LRL - atr_pulse_width,msec)]
    AOO.AOO_Pace -> AOO.AOO_Charge : [after(atr_pulse_width,msec)]
  (default) -> Start
  Start -> VVIR [order 8] : [mode == 8]
  VVIR -> Start : [mode ~= 8]
  Start -> VVI [order 6] : [mode == 4]
  VVI -> Start : [mode ~= 4]
  Start -> AAIR [order 7] : [mode == 7]
  AAIR -> Start : [mode ~= 7]
  Start -> AAI [order 5] : [mode == 3]
  AAI -> Start : [mode ~= 3]
  Start -> VOOR [order 4] : [mode == 6]
  Start -> VOO [order 1] : [mode == 2]
  VOO -> Start : [mode ~= 2]
  VOOR -> Start : [mode ~= 6]
  AOOR -> Start : [mode ~= 5]
  AOO -> Start : [mode ~= 1]
  Start -> AOO [order 2] : [mode == 1]
  Start -> AOOR [order 3] : [mode == 5]
  data: PACE_CHARGE_CTRL output; VENT_CMP_REF_PWM output; Z_ATR_CTRL output; PACING_REF_PWM output; ATR_CMP_REF_PWM output; Z_VENT_CTRL output; mode input; ATR_PACE_CTRL output; VENT_PACE_CTRL output; PACE_GND_CTRL output; atr_amp input; ATR_GND_CTRL output; atr_pulse_width input; LRL input; vent_amp input; VENT_GND_CTRL output; vent_pulse_width input; FRONTEND_CTRL output; atr_sense_amp input; ARP input; ATR_CMP_DETECT input; vent_sense_amp input; VRP input; VENT_CMP_DETECT input; URL input; modulated_period input
